simulink model "afe_inv_psm_param"  (R2026b)
settings: Solver=ode23t  StopTime=param.sim.simlength  FixedStep=tc  MaxStep=param.glb_time.tc  RelTol=1e-4
values from neighbouring files (symbols this model uses):
  param = add_template_extras(param, options)    [init_model.m]
undefined symbols (not defined in the file or in its folder): magnitude, omega_m_bez
libraries: fl_lib x330, nesl_utility x174, igbt_simple_2th_lib x12, moving_average_filter x10, moving_average_filter_cc x8, sl_discontinuities x3, single_phase_transformer_lib x3, linear_double_integrator_observer_ccaller x2, discrete_time_low_pass_filter x2, threephase_inductor_lib x2, three_phase_pwm_modulator x2, three_phase_inverter_ideal_switch_based_model x2
(part 3 of 13)

== system afe_inv_psm_param/afe_abc_inv_psm_mod1/afe/three_phase_inverter_igbt_based_with_thermal_model ==
  gate_commands : Inport
  Bus Selector : BusSelector  OutputSignals=module_1.igbt_ploss_Q2,module_1.igbt_voltage_Q2,module_1.igbt_current_Q2,module_1.igbt_JH_temp_Q2,module_1.igbt_HA_temp_Q2
  Bus Selector1 : BusSelector  OutputSignals=module_1.igbt_ploss_Q1,module_1.igbt_voltage_Q1,module_1.igbt_current_Q1,module_1.igbt_JH_temp_Q1,module_1.igbt_HA_temp_Q1
  Bus Selector2 : BusSelector  OutputSignals=module_2.igbt_ploss_Q3,module_2.igbt_voltage_Q3,module_2.igbt_current_Q3,module_2.igbt_JH_temp_Q3,module_2.igbt_HA_temp_Q3
  Bus Selector3 : BusSelector  OutputSignals=module_1.diode_ploss_Q1,module_1.diode_JH_temp_Q1,module_1.diode_HA_temp_Q1,module_1.diode_current_Q1
  three_phase_inverter_with_igbt_simple_2th : Subsystem  mask{vce_sat_m=param.afe.igbt.Vce_sat, v_gamma_m=param.afe.igbt.Vdon_diode, Vth_gate_m=param.afe.igbt.Vth, Vth_gate_hyst_m=0.85, Eon_m=param.afe.igbt.Eon*1000, Eoff_m=param.afe.igbt.Eoff*1000, Err_m=param.afe.igbt.Erec*1000, Ic_ref_m=param.afe.igbt.Ion_sw_losses, Vdc_ref_m=param.afe.igbt.Voff_sw_losses, Vblock_Errf_m=50, rce_on_m=param.afe.igbt.Rce_on*1000, rd_on_m=param.afe.igbt.Rdon_diode*1000, Gce_off_m=1e-6, time_constant_edge_m=param.glb_time.tc, time_constant_ploss_m=1e3, Csnubber_m=param.afe.igbt.Csnubber, Rsnubber_m=param.afe.igbt.Rsnubber, rth_switch_JH_m=param.afe.igbt.Rth_switch_JH, rth_switch_HA_m=param.thermal.heatsink.Rth_switch_HA, rth_diode_JH_m=param.afe.igbt.Rth_diode_JH, rth_diode_HA_m=param.thermal.heatsink.Rth_diode_HA, JunctionTermalMass_m=param.afe.igbt.JunctionTermalMass, Tambient_m=param.thermal.Tambient, mass_heatsink_m=param.thermal.heatsink.no_weight, specific_heat_m=param.thermal.heatsink.cp}
      mask prompts: vce_sat_m "Collector-emitter on-stage voltage [V]"; v_gamma_m "Diode forward voltage [V]"; Vth_gate_m "Gate-emitter threshold voltage [V]"; Vth_gate_hyst_m "Half hysteresis band for the switching events [V]"; Eon_m "Turn-on energy at Ic_ref, Vdc_ref [mJ]"; Eoff_m "Turn-off energy at Ic_ref, Vdc_ref [mJ]"; Err_m "Reverse recovery energy at Ic_ref, Vdc_ref [mJ]"; Ic_ref_m "Reference current of the energies [A]"; Vdc_ref_m "Reference voltage of the energies [V]"; Vblock_Errf_m "V block Err"; rce_on_m "IGBT on-state series resistance [mOhm]"; rd_on_m "Diode series resistance [mOhm]"; Gce_off_m "Off-state conductance [1/Ohm]"; time_constant_edge_m "Sample&hold time constant (<< on-time) [us]"; time_constant_ploss_m "Loss averaging time constant (2-5 x Tsw) [us]"; Csnubber_m "Csnubber [F]"; Rsnubber_m "Rsnubber [Ohm]"; rth_switch_JH_m "Thermal impedance Junction-heatsink switch [K/W]"; rth_switch_HA_m "Thermal impedance heatsink-ambient switch[K/W]"; rth_diode_JH_m "Thermal impedance Junction-heatsink diode [K/W]"; rth_diode_HA_m "Thermal impedance heatsink-ambient diode [K/W]"; JunctionTermalMass_m "Junction Thermal Mass [J/K]"; Tambient_m "Ambient temperature [degC]"; mass_heatsink_m "Mass heatsink [kg]"; specific_heat_m "Specific heat capacity of the heatsink [J/K/Kg]"
  udc(+) : PMIOPort  Side=Left
  u : PMIOPort  Port=2  Side=Right
  v : PMIOPort  Port=3  Side=Right
  udc(-) : PMIOPort  Port=4  Side=Left
  w : PMIOPort  Port=5  Side=Right
  tag scope: diode_HA_temp_afeQ1=global, diode_JH_temp_afeQ1=global, diode_current_afeQ1=global, diode_ploss_afeQ1=global, igbt_HA_temp_afeQ1=global, igbt_HA_temp_afeQ2=global, igbt_HA_temp_afeQ3=global, igbt_JH_temp_afeQ1=global, igbt_JH_temp_afeQ2=global, igbt_JH_temp_afeQ3=global, igbt_current_afeQ1=global, igbt_current_afeQ2=global, igbt_current_afeQ3=global, igbt_ploss_afeQ1=global, igbt_ploss_afeQ2=global, igbt_ploss_afeQ3=global, igbt_voltage_afeQ1=global, igbt_voltage_afeQ2=global, igbt_voltage_afeQ3=global
  wires:
  gate_commands/1 -> three_phase_inverter_with_igbt_simple_2th/1(gate_commands)
  Bus Selector3/3 -> [diode_HA_temp_afeQ1]  "<diode_HA_temp_Q1>"
  Bus Selector/1 -> [igbt_ploss_afeQ2]  "<igbt_ploss_Q2>"
  Bus Selector3/2 -> [diode_JH_temp_afeQ1]  "<diode_JH_temp_Q1>"
  Bus Selector1/2 -> [igbt_voltage_afeQ1]  "<igbt_voltage_Q1>"
  Bus Selector/2 -> [igbt_voltage_afeQ2]  "<igbt_voltage_Q2>"
  Bus Selector/5 -> [igbt_HA_temp_afeQ2]  "<igbt_HA_temp_Q2>"
  Bus Selector2/5 -> [igbt_HA_temp_afeQ3]  "<igbt_HA_temp_Q3>"
  Bus Selector2/2 -> [igbt_voltage_afeQ3]  "<igbt_voltage_Q3>"
  Bus Selector/4 -> [igbt_JH_temp_afeQ2]  "<igbt_JH_temp_Q2>"
  Bus Selector1/4 -> [igbt_JH_temp_afeQ1]  "<igbt_JH_temp_Q1>"
  Bus Selector3/1 -> [diode_ploss_afeQ1]  "<diode_ploss_Q1>"
  Bus Selector2/4 -> [igbt_JH_temp_afeQ3]  "<igbt_JH_temp_Q3>"
  Bus Selector2/3 -> [igbt_current_afeQ3]  "<igbt_current_Q3>"
  three_phase_inverter_with_igbt_simple_2th/1(m) -> Bus Selector3/1, Bus Selector2/1, Bus Selector/1, Bus Selector1/1
  Bus Selector1/3 -> [igbt_current_afeQ1]  "<igbt_current_Q1>"
  Bus Selector/3 -> [igbt_current_afeQ2]  "<igbt_current_Q2>"
  Bus Selector1/5 -> [igbt_HA_temp_afeQ1]  "<igbt_HA_temp_Q1>"
  Bus Selector2/1 -> [igbt_ploss_afeQ3]  "<igbt_ploss_Q3>"
  Bus Selector1/1 -> [igbt_ploss_afeQ1]  "<igbt_ploss_Q1>"
  Bus Selector3/4 -> [diode_current_afeQ1]  "<diode_current_Q1>"
  connections:
  u/RConn1 -- three_phase_inverter_with_igbt_simple_2th/RConn1
  v/RConn1 -- three_phase_inverter_with_igbt_simple_2th/RConn2
  udc(-)/RConn1 -- three_phase_inverter_with_igbt_simple_2th/LConn2
  udc(+)/RConn1 -- three_phase_inverter_with_igbt_simple_2th/LConn1
  w/RConn1 -- three_phase_inverter_with_igbt_simple_2th/RConn3

== system afe_inv_psm_param/afe_abc_inv_psm_mod1/afe/three_phase_inverter_mosfet_based_with_thermal_model ==
  gate_commands : Inport
  Bus Selector : BusSelector  OutputSignals=mosfet_ploss_Q2,mosfet_voltage_Q2,mosfet_current_Q2,mosfet_JH_temp_Q2,mosfet_HA_temp_Q2
  Bus Selector1 : BusSelector  OutputSignals=mosfet_ploss_Q1,mosfet_voltage_Q1,mosfet_current_Q1,mosfet_JH_temp_Q1,mosfet_HA_temp_Q1
  Bus Selector2 : BusSelector  OutputSignals=mosfet_ploss_Q3,mosfet_voltage_Q3,mosfet_current_Q3,mosfet_JH_temp_Q3,mosfet_HA_temp_Q3
  three phase inverter mosfet based with thermal model : three_phase_inverter_mosfet_based_with_thermal_model/three phase inverter mosfet based with thermal model  mass_heatsink_m=0.2  specific_heat_m=880  rth_mosfet_HA_m=0.02  rth_mosfet_JH_m=0.075  Rds_on_m=0.00185  Vth_m=7.5  Eon_m=0.077  Eoff_m=0.108  Voff_sw_loss_m=1300  Ion_sw_loss_m=1000  Vdon_diode_m=4  Rdon_diode_m=0.00185  JunctionTermalMass_m=2  Tambient_m=40  DThs_init_m=0
  u : PMIOPort  Side=Right
  udc(+) : PMIOPort  Port=2  Side=Left
  v : PMIOPort  Port=3  Side=Right
  udc(-) : PMIOPort  Port=4  Side=Left
  w : PMIOPort  Port=5  Side=Right
  tag scope: mosfet_HA_temp_afeQ1=global, mosfet_HA_temp_afeQ2=global, mosfet_HA_temp_afeQ3=global, mosfet_JH_temp_afeQ1=global, mosfet_JH_temp_afeQ2=global, mosfet_JH_temp_afeQ3=global, mosfet_current_afeQ1=global, mosfet_current_afeQ2=global, mosfet_current_afeQ3=global, mosfet_ploss_afeQ1=global, mosfet_ploss_afeQ2=global, mosfet_ploss_afeQ3=global, mosfet_voltage_afeQ1=global, mosfet_voltage_afeQ2=global, mosfet_voltage_afeQ3=global
  wires:
  gate_commands/1 -> three phase inverter mosfet based with thermal model/1
  three phase inverter mosfet based with thermal model/1 -> Bus Selector/1, Bus Selector2/1, Bus Selector1/1
  Bus Selector2/1 -> [mosfet_ploss_afeQ3]  "<mosfet_ploss_Q3>"
  Bus Selector2/2 -> [mosfet_voltage_afeQ3]  "<mosfet_voltage_Q3>"
  Bus Selector2/3 -> [mosfet_current_afeQ3]  "<mosfet_current_Q3>"
  Bus Selector2/5 -> [mosfet_HA_temp_afeQ3]  "<mosfet_HA_temp_Q3>"
  Bus Selector2/4 -> [mosfet_JH_temp_afeQ3]  "<mosfet_JH_temp_Q3>"
  Bus Selector/1 -> [mosfet_ploss_afeQ2]  "<mosfet_ploss_Q2>"
  Bus Selector/2 -> [mosfet_voltage_afeQ2]  "<mosfet_voltage_Q2>"
  Bus Selector/3 -> [mosfet_current_afeQ2]  "<mosfet_current_Q2>"
  Bus Selector/4 -> [mosfet_JH_temp_afeQ2]  "<mosfet_JH_temp_Q2>"
  Bus Selector/5 -> [mosfet_HA_temp_afeQ2]  "<mosfet_HA_temp_Q2>"
  Bus Selector1/1 -> [mosfet_ploss_afeQ1]  "<mosfet_ploss_Q1>"
  Bus Selector1/2 -> [mosfet_voltage_afeQ1]  "<mosfet_voltage_Q1>"
  Bus Selector1/3 -> [mosfet_current_afeQ1]  "<mosfet_current_Q1>"
  Bus Selector1/4 -> [mosfet_JH_temp_afeQ1]  "<mosfet_JH_temp_Q1>"
  Bus Selector1/5 -> [mosfet_HA_temp_afeQ1]  "<mosfet_HA_temp_Q1>"
  connections:
  three phase inverter mosfet based with thermal model/RConn3 -- w/RConn1
  three phase inverter mosfet based with thermal model/RConn2 -- v/RConn1
  three phase inverter mosfet based with thermal model/LConn1 -- udc(+)/RConn1
  three phase inverter mosfet based with thermal model/LConn2 -- udc(-)/RConn1
  three phase inverter mosfet based with thermal model/RConn1 -- u/RConn1

== system afe_inv_psm_param/afe_abc_inv_psm_mod1/battery/single_phase_ui_measure ==
  Bus Creator : BusCreator  Inputs=2
  Current Sensor : fl_lib/Electrical/Electrical Sensors/Current Sensor
  Selector : Selector  InputPortWidth=2  IndexOptions=Index vector (dialog)  Indices=2  OutputSizes=1  RuntimeRangeChecks=off
  Selector1 : Selector  InputPortWidth=2  IndexOptions=Index vector (dialog)  Indices=1  OutputSizes=1  RuntimeRangeChecks=off
  Voltage Sensor : fl_lib/Electrical/Electrical Sensors/Voltage Sensor
  dab input modA : Scope  NumInputPorts=2
      settings: ActiveDisplayYMinimum=-413.54291450338707  ActiveDisplayYMaximum=396.93489435257015  DataLoggingVariableName=ScopeData2
  iph : nesl_utility/PS-Simulink Converter  PhysicalDomain=network_engine_domain  SubClassName=ps_output  LeftPortType=input  RightPortType=output  PseudoPeriodic=off  Frequencies=[]  VectorFormat=1-D array  Unit=A  AffineConversion=off
  uph : nesl_utility/PS-Simulink Converter  PhysicalDomain=network_engine_domain  SubClassName=ps_output  LeftPortType=input  RightPortType=output  PseudoPeriodic=off  Frequencies=[]  VectorFormat=1-D array  Unit=V  AffineConversion=off
  Udc(+) : PMIOPort  Side=Left
  udc(+) : PMIOPort  Port=2  Side=Right
  Udc(-) : PMIOPort  Port=3  Side=Left
  udc(-) : PMIOPort  Port=4  Side=Right
  tag scope: current_battery=global, voltage_battery=global
  wires:
  Bus Creator/1 -> Selector/1, Selector1/1  "ui_data"
  iph/1 -> Bus Creator/1  "iph"
  uph/1 -> Bus Creator/2  "uph"
  Selector1/1 -> [current_battery], dab input modA/1  "current_battery"
  Selector/1 -> dab input modA/2, [voltage_battery]  "voltage_battery"
  connections:
  iph/LConn1 -- Current Sensor/RConn1
  Voltage Sensor/LConn1 -- Current Sensor/LConn1 -- Udc(+)/RConn1
  Current Sensor/RConn2 -- udc(+)/RConn1
  Voltage Sensor/RConn1 -- uph/LConn1
  Voltage Sensor/RConn2 -- Udc(-)/RConn1 -- udc(-)/RConn1

== system afe_inv_psm_param/afe_abc_inv_psm_mod1/brake/Rbrake ==
  PS-Simulink Converter2 : nesl_utility/PS-Simulink Converter  PhysicalDomain=network_engine_domain  SubClassName=ps_output  LeftPortType=input  RightPortType=output  PseudoPeriodic=off  Frequencies=[]  VectorFormat=1-D array  Unit=degC  AffineConversion=off
  PS-Simulink Converter3 : nesl_utility/PS-Simulink Converter  PhysicalDomain=network_engine_domain  SubClassName=ps_output  LeftPortType=input  RightPortType=output  PseudoPeriodic=off  Frequencies=[]  VectorFormat=1-D array  Unit=W  AffineConversion=off
  Rbrake_thermal : Scope  NumInputPorts=2
      settings: ActiveDisplayYMinimum=-0.005623823950706707  ActiveDisplayYMaximum=0.05061441555636037  DataLoggingVariableName=ScopeData33
  Resistor1 : ee_lib/Passive/Resistor  R=param.afe.hw.Rbrake Ohm  enable_R_tol=ee.enum.toleranceApplication.none  R_tol=5  tol_distribution=ee.enum.toleranceDistribution.uniform  nSigma=4  enable_operating_limits=ee.enum.enable.no  operating_limit_action=ee.enum.passive.reportOpLim.warn  power_rating=1 W  max_working_voltage=100 V  noise_mode=ee.enum.sources.noise.Disabled  Tdevice=25 degC  sample_time=1e-3 s  repeatability=ee.enum.ic.repeatability.notRepeatable  user_seed=0  auto_seed=3499211588  power_derating_T1=70 degC  power_derating_T2=155 degC  operating_temperature_range_vec=[-50, 150] degC  alpha=3.93e-3 1/K  Tmeas=25 degC  thermal_mass=100 J/K  temperature_specify=off  temperature_priority=High  temperature=298.15 K  temperature_nominal_specify=off  temperature_nominal_value=1  temperature_nominal_unit=K
  Tambient : fl_lib/Thermal/Thermal Sources/Temperature Source  temperature=param.thermal.Tambient degC
  Temperature Sensor1 : fl_lib/Thermal/Thermal Sensors/Temperature Sensor  temperature_measure=foundation.enum.MeasurementReference.difference
  To Workspace1 : ToWorkspace  VariableName=RbrakePowerFlow_mod1_sim  SampleTime=param.glb_time.tc
      settings: MaxDataPoints=param.glb_time.Nc
  To Workspace10 : ToWorkspace  VariableName=RbrakeTemperature_mod1_sim  SampleTime=param.glb_time.tc
      settings: MaxDataPoints=param.glb_time.Nc
  heatsink_C : fl_lib/Thermal/Thermal Elements/Thermal Mass  mass_type=foundation.enum.constant_variable.constant  mass=40 kg  sp_heat=505 J/(K*kg)  mass_min=1e-6 kg  num_ports=foundation.enum.numPorts2.one  m_specify=off  m_priority=High  m=1 kg  m_nominal_specify=off  m_nominal_value=1  m_nominal_unit=kg  T_specify=on  T_priority=High  T=param.thermal.DThs_init+param.thermal.Tambient degC  T_nominal_specify=off  T_nominal_value=1  T_nominal_unit=K  Q_specify=off  Q_priority=High  Q=0 W  Q_nominal_specify=off  Q_nominal_value=1  Q_nominal_unit=W
  power_losses_switch : fl_lib/Thermal/Thermal Sensors/Heat Flow Rate Sensor
  switch_heatsink : fl_lib/Thermal/Thermal Elements/Thermal Resistance  resistance=300/48e3 K/W  T_specify=off  T_priority=High  T=0 deltadegC  T_nominal_specify=off  T_nominal_value=1  T_nominal_unit=K  Q_specify=off  Q_priority=None  Q=0 W  Q_nominal_specify=off  Q_nominal_value=1  Q_nominal_unit=W
  A : PMIOPort  Side=Left
  B : PMIOPort  Port=2  Side=Right
  wires:
  PS-Simulink Converter2/1 -> To Workspace10/1, Rbrake_thermal/1  "RbrakeTemperature"
  PS-Simulink Converter3/1 -> To Workspace1/1, Rbrake_thermal/2  "RbrakePowerFlow"
  connections:
  Resistor1/LConn1 -- A/RConn1
  Resistor1/RConn1 -- B/RConn1
  Tambient/LConn1 -- Temperature Sensor1/RConn1 -- switch_heatsink/RConn1
  Temperature Sensor1/LConn1 -- power_losses_switch/RConn2 -- heatsink_C/LConn1 -- switch_heatsink/LConn1
  Temperature Sensor1/RConn2 -- PS-Simulink Converter2/LConn1
  power_losses_switch/LConn1 -- Resistor1/LConn2
  power_losses_switch/RConn1 -- PS-Simulink Converter3/LConn1

== system afe_inv_psm_param/afe_abc_inv_psm_mod1/brake/switch_1 ==
  Capacitor : fl_lib/Electrical/Electrical Elements/Capacitor  c=param.afe.ideal_switch.Csnubber F  r=param.afe.ideal_switch.Rsnubber Ohm  g=0 1/Ohm  i_specify=off  i_priority=None  i=0 A  i_nominal_specify=off  i_nominal_value=1  i_nominal_unit=A  v_specify=off  v_priority=None  v=0 V  v_nominal_specify=off  v_nominal_value=1  v_nominal_unit=V  vc_specify=off  vc_priority=High  vc=0 V  vc_nominal_specify=off  vc_nominal_value=1  vc_nominal_unit=V
  Diode : fl_lib/Electrical/Electrical Elements/Diode  Vf=param.afe.ideal_switch.Vgamma V  Ron=param.afe.ideal_switch.Rdon_diode Ohm  Goff=1e-8 1/Ohm  i_specify=off  i_priority=None  i=0 A  i_nominal_specify=off  i_nominal_value=1  i_nominal_unit=A  v_specify=off  v_priority=None  v=0 V  v_nominal_specify=off  v_nominal_value=1  v_nominal_unit=V
  C : PMIOPort  Side=Left
  E : PMIOPort  Port=2  Side=Right
  connections:
  Diode/LConn1 -- Capacitor/RConn1 -- E/RConn1
  Diode/RConn1 -- C/RConn1 -- Capacitor/LConn1

== system afe_inv_psm_param/afe_abc_inv_psm_mod1/brake/switch_2 ==
  Capacitor : fl_lib/Electrical/Electrical Elements/Capacitor  c=param.afe.ideal_switch.Csnubber F  r=param.afe.ideal_switch.Rsnubber Ohm  g=0 1/Ohm  i_specify=off  i_priority=None  i=0 A  i_nominal_specify=off  i_nominal_value=1  i_nominal_unit=A  v_specify=off  v_priority=None  v=0 V  v_nominal_specify=off  v_nominal_value=1  v_nominal_unit=V  vc_specify=off  vc_priority=High  vc=0 V  vc_nominal_specify=off  vc_nominal_value=1  vc_nominal_unit=V
  Diode : fl_lib/Electrical/Electrical Elements/Diode  Vf=param.afe.ideal_switch.Vgamma V  Ron=param.afe.ideal_switch.Rdon_diode Ohm  Goff=1e-8 1/Ohm  i_specify=off  i_priority=None  i=0 A  i_nominal_specify=off  i_nominal_value=1  i_nominal_unit=A  v_specify=off  v_priority=None  v=0 V  v_nominal_specify=off  v_nominal_value=1  v_nominal_unit=V
  Switch : fl_lib/Electrical/Electrical Elements/Switch  R_closed=param.afe.ideal_switch.Rds_on Ohm  G_open=1e-8 1/Ohm  Threshold=7.5  i_specify=off  i_priority=None  i=0 A  i_nominal_specify=off  i_nominal_value=1  i_nominal_unit=A  v_specify=off  v_priority=None  v=0 V  v_nominal_specify=off  v_nominal_value=1  v_nominal_unit=V
  G : PMIOPort  Side=Left
  C : PMIOPort  Port=2  Side=Left
  E : PMIOPort  Port=3  Side=Right
  connections:
  Switch/RConn2 -- C/RConn1 -- Capacitor/LConn1 -- Diode/RConn1
  Switch/RConn1 -- G/RConn1
  Switch/LConn1 -- E/RConn1 -- Capacitor/RConn1 -- Diode/LConn1

== system afe_inv_psm_param/afe_abc_inv_psm_mod1/inverter/inverter ==
  gate_cmds_uvw : Inport
  sv_pwm : Subsystem
  three_phase_inverter_ideal_switch_based_model : Subsystem  Commented=on
  three_phase_inverter_igbt_based_with_thermal_model : Subsystem
  three_phase_inverter_mosfet_based_with_thermal_model : Subsystem  Commented=on
  u : PMIOPort  Side=Left
  v : PMIOPort  Port=2  Side=Left
  w : PMIOPort  Port=3  Side=Left
  udc(+) : PMIOPort  Port=4  Side=Right
  udc(-) : PMIOPort  Port=5  Side=Right
  wires:
  sv_pwm/1(gate_cmds) -> three_phase_inverter_mosfet_based_with_thermal_model/1(gate_commands), three_phase_inverter_igbt_based_with_thermal_model/1(gate_commands), three_phase_inverter_ideal_switch_based_model/1(gate_commands)
  gate_cmds_uvw/1 -> sv_pwm/1(gate_cmds_uvw)
  connections:
  udc(+)/RConn1 -- three_phase_inverter_ideal_switch_based_model/LConn1 -- three_phase_inverter_igbt_based_with_thermal_model/LConn1 -- three_phase_inverter_mosfet_based_with_thermal_model/LConn1
  udc(-)/RConn1 -- three_phase_inverter_ideal_switch_based_model/LConn2 -- three_phase_inverter_igbt_based_with_thermal_model/LConn2 -- three_phase_inverter_mosfet_based_with_thermal_model/LConn2
  u/RConn1 -- three_phase_inverter_igbt_based_with_thermal_model/RConn1 -- three_phase_inverter_ideal_switch_based_model/RConn1 -- three_phase_inverter_mosfet_based_with_thermal_model/RConn1
  v/RConn1 -- three_phase_inverter_igbt_based_with_thermal_model/RConn2 -- three_phase_inverter_ideal_switch_based_model/RConn2 -- three_phase_inverter_mosfet_based_with_thermal_model/RConn2
  w/RConn1 -- three_phase_inverter_igbt_based_with_thermal_model/RConn3 -- three_phase_inverter_ideal_switch_based_model/RConn3 -- three_phase_inverter_mosfet_based_with_thermal_model/RConn3

== system afe_inv_psm_param/grid/grid_emulator/3ph_Dyg ==
  Electrical Reference1 : fl_lib/Electrical/Electrical Elements/Electrical Reference
  ph1 : single_phase_transformer_lib/single phase transformer  Lm=param.grid.emu.trafo.Lm1 H  n1=param.grid.emu.trafo.n1  n2=param.grid.emu.trafo.n2  Rd1=param.grid.emu.trafo.Rd1 Ohm  Rd2=param.grid.emu.trafo.Rd2 Ohm  Ld1=param.grid.emu.trafo.Ld1 H  Ld2=param.grid.emu.trafo.Ld2 H  Rfe=param.grid.emu.trafo.Rfe1 Ohm  phi_specify=off  phi_priority=None  phi=0 V*s  phi_nominal_specify=off  phi_nominal_value=1  phi_nominal_unit=V*s  i1_specify=off  i1_priority=None  i1=0 A  i1_nominal_specify=off  i1_nominal_value=1  i1_nominal_unit=A  i2_specify=off  i2_priority=None  i2=0 A  i2_nominal_specify=off  i2_nominal_value=1  i2_nominal_unit=A  ife_specify=off  ife_priority=None  ife=0 A  ife_nominal_specify=off  ife_nominal_value=1  ife_nominal_unit=A  u1_specify=off  u1_priority=None  u1=0 V  u1_nominal_specify=off  u1_nominal_value=1  u1_nominal_unit=V  u2_specify=off  u2_priority=None  u2=0 V  u2_nominal_specify=off  u2_nominal_value=1  u2_nominal_unit=V
  ph2 : single_phase_transformer_lib/single phase transformer  Lm=param.grid.emu.trafo.Lm1 H  n1=param.grid.emu.trafo.n1  n2=param.grid.emu.trafo.n2  Rd1=param.grid.emu.trafo.Rd1 Ohm  Rd2=param.grid.emu.trafo.Rd2 Ohm  Ld1=param.grid.emu.trafo.Ld1 H  Ld2=param.grid.emu.trafo.Ld2 H  Rfe=param.grid.emu.trafo.Rfe1 Ohm  phi_specify=off  phi_priority=None  phi=0 V*s  phi_nominal_specify=off  phi_nominal_value=1  phi_nominal_unit=V*s  i1_specify=off  i1_priority=None  i1=0 A  i1_nominal_specify=off  i1_nominal_value=1  i1_nominal_unit=A  i2_specify=off  i2_priority=None  i2=0 A  i2_nominal_specify=off  i2_nominal_value=1  i2_nominal_unit=A  ife_specify=off  ife_priority=None  ife=0 A  ife_nominal_specify=off  ife_nominal_value=1  ife_nominal_unit=A  u1_specify=off  u1_priority=None  u1=0 V  u1_nominal_specify=off  u1_nominal_value=1  u1_nominal_unit=V  u2_specify=off  u2_priority=None  u2=0 V  u2_nominal_specify=off  u2_nominal_value=1  u2_nominal_unit=V
  ph3 : single_phase_transformer_lib/single phase transformer  Lm=param.grid.emu.trafo.Lm1 H  n1=param.grid.emu.trafo.n1  n2=param.grid.emu.trafo.n2  Rd1=param.grid.emu.trafo.Rd1 Ohm  Rd2=param.grid.emu.trafo.Rd2 Ohm  Ld1=param.grid.emu.trafo.Ld1 H  Ld2=param.grid.emu.trafo.Ld2 H  Rfe=param.grid.emu.trafo.Rfe1 Ohm  phi_specify=off  phi_priority=None  phi=0 V*s  phi_nominal_specify=off  phi_nominal_value=1  phi_nominal_unit=V*s  i1_specify=off  i1_priority=None  i1=0 A  i1_nominal_specify=off  i1_nominal_value=1  i1_nominal_unit=A  i2_specify=off  i2_priority=None  i2=0 A  i2_nominal_specify=off  i2_nominal_value=1  i2_nominal_unit=A  ife_specify=off  ife_priority=None  ife=0 A  ife_nominal_specify=off  ife_nominal_value=1  ife_nominal_unit=A  u1_specify=off  u1_priority=None  u1=0 V  u1_nominal_specify=off  u1_nominal_value=1  u1_nominal_unit=V  u2_specify=off  u2_priority=None  u2=0 V  u2_nominal_specify=off  u2_nominal_value=1  u2_nominal_unit=V
  ua : PMIOPort  Side=Right
  ub : PMIOPort  Port=2  Side=Right
  uc : PMIOPort  Port=3  Side=Right
  Ua : PMIOPort  Port=4  Side=Left
  Ub : PMIOPort  Port=5  Side=Left
  Uc : PMIOPort  Port=6  Side=Left
  connections:
  Electrical Reference1/LConn1 -- ph3/RConn2 -- ph2/RConn2 -- ph1/RConn2
  ph3/RConn1 -- uc/RConn1
  ph1/LConn1 -- ph3/LConn2 -- Ua/RConn1
  ph1/RConn1 -- ua/RConn1
  ph2/RConn1 -- ub/RConn1
  ph1/LConn2 -- ph2/LConn1 -- Ub/RConn1
  Uc/RConn1 -- ph3/LConn1 -- ph2/LConn2

== system afe_inv_psm_param/grid/grid_emulator/threephase_vi_measures ==
  Bus Creator : BusCreator  Inputs=6
  Current Sensor : fl_lib/Electrical/Electrical Sensors/Current Sensor
  Current Sensor1 : fl_lib/Electrical/Electrical Sensors/Current Sensor
  Current Sensor2 : fl_lib/Electrical/Electrical Sensors/Current Sensor
  Electrical Reference1 : fl_lib/Electrical/Electrical Elements/Electrical Reference
  Voltage Sensor : fl_lib/Electrical/Electrical Sensors/Voltage Sensor
  Voltage Sensor1 : fl_lib/Electrical/Electrical Sensors/Voltage Sensor
  Voltage Sensor2 : fl_lib/Electrical/Electrical Sensors/Voltage Sensor
  i : Selector  InputPortWidth=6  IndexOptions=Index vector (dialog)  Indices=[4 5 6]  OutputSizes=1  RuntimeRangeChecks=off
  ia_grid : nesl_utility/PS-Simulink Converter  PhysicalDomain=network_engine_domain  SubClassName=ps_output  LeftPortType=input  RightPortType=output  PseudoPeriodic=off  Frequencies=[]  VectorFormat=1-D array  Unit=A  AffineConversion=off
  ib_grid : nesl_utility/PS-Simulink Converter  PhysicalDomain=network_engine_domain  SubClassName=ps_output  LeftPortType=input  RightPortType=output  PseudoPeriodic=off  Frequencies=[]  VectorFormat=1-D array  Unit=A  AffineConversion=off
  ic_grid : nesl_utility/PS-Simulink Converter  PhysicalDomain=network_engine_domain  SubClassName=ps_output  LeftPortType=input  RightPortType=output  PseudoPeriodic=off  Frequencies=[]  VectorFormat=1-D array  Unit=A  AffineConversion=off
  u : Selector  InputPortWidth=6  IndexOptions=Index vector (dialog)  Indices=[1 2 3]  OutputSizes=1  RuntimeRangeChecks=off
  ua_grid : nesl_utility/PS-Simulink Converter  PhysicalDomain=network_engine_domain  SubClassName=ps_output  LeftPortType=input  RightPortType=output  PseudoPeriodic=off  Frequencies=[]  VectorFormat=1-D array  Unit=V  AffineConversion=off
  ub_grid : nesl_utility/PS-Simulink Converter  PhysicalDomain=network_engine_domain  SubClassName=ps_output  LeftPortType=input  RightPortType=output  PseudoPeriodic=off  Frequencies=[]  VectorFormat=1-D array  Unit=V  AffineConversion=off
  uc_grid : nesl_utility/PS-Simulink Converter  PhysicalDomain=network_engine_domain  SubClassName=ps_output  LeftPortType=input  RightPortType=output  PseudoPeriodic=off  Frequencies=[]  VectorFormat=1-D array  Unit=V  AffineConversion=off
  Ua : PMIOPort  Side=Left
  ua : PMIOPort  Port=2  Side=Right
  Ub : PMIOPort  Port=3  Side=Left
  ub : PMIOPort  Port=4  Side=Right
  Uc : PMIOPort  Port=5  Side=Left
  uc : PMIOPort  Port=6  Side=Right
  tag scope: i_abc_line=global, u_abc_line=global
  wires:
  Bus Creator/1 -> i/1, u/1  "vi_data"
  ib_grid/1 -> Bus Creator/5  "ib"
  ia_grid/1 -> Bus Creator/4  "ia"
  ic_grid/1 -> Bus Creator/6  "ic"
  ua_grid/1 -> Bus Creator/1  "ua"
  ub_grid/1 -> Bus Creator/2  "ub"
  uc_grid/1 -> Bus Creator/3  "uc"
  i/1 -> [i_abc_line]
  u/1 -> [u_abc_line]
  connections:
  Current Sensor1/LConn1 -- Ub/RConn1 -- Voltage Sensor1/LConn1
  Electrical Reference1/LConn1 -- Voltage Sensor/RConn2 -- Voltage Sensor2/RConn2 -- Voltage Sensor1/RConn2
  Voltage Sensor/RConn1 -- ua_grid/LConn1
  Current Sensor/RConn2 -- ua/RConn1
  Voltage Sensor1/RConn1 -- ub_grid/LConn1
  Voltage Sensor2/LConn1 -- Current Sensor2/LConn1 -- Uc/RConn1
  Current Sensor/LConn1 -- Ua/RConn1 -- Voltage Sensor/LConn1
  Current Sensor1/RConn2 -- ub/RConn1
  Voltage Sensor2/RConn1 -- uc_grid/LConn1
  ib_grid/LConn1 -- Current Sensor1/RConn1
  ia_grid/LConn1 -- Current Sensor/RConn1
  ic_grid/LConn1 -- Current Sensor2/RConn1
  Current Sensor2/RConn2 -- uc/RConn1

== system afe_inv_psm_param/afe_abc_inv_psm_mod1/AFE_control/afe_control/FRT-VDE4110 ==
  Constant : Constant  Value=0
  FRT-Detection : Subsystem
  FRT-PosNegReactiveCurrentReferences : Subsystem
  Terminator : Terminator
  Terminator1 : Terminator
  frt_detection_output : Scope  NumInputPorts=3
      settings: ActiveDisplayYMinimum=-0.12499999999999997  ActiveDisplayYMaximum=1.125
  tag scope: frt_active=scoped, pwr_lim_enable=scoped
  wires:
  [v_grid_pos_xi_avg] -> FRT-PosNegReactiveCurrentReferences/1(In1)
  [v_grid_neg_xi_avg] -> FRT-PosNegReactiveCurrentReferences/3(In3)
  [v_grid_neg_eta_avg] -> FRT-PosNegReactiveCurrentReferences/4(In4)
  [v_grid_pos_eta_avg] -> FRT-PosNegReactiveCurrentReferences/2(In2)
  FRT-Detection/4(frt_active) -> frt_detection_output/2, [frt_active]  "frt_active"
  FRT-Detection/5(pwr_lim_enable) -> frt_detection_output/3, [pwr_lim_enable]  "pwr_lim_enable"
  FRT-Detection/2(frt_state) -> frt_detection_output/1  "frt_state"
  Constant/1 -> FRT-Detection/1(red_dyn_enabled)
  FRT-Detection/1(frt_exceeded) -> Terminator/1
  FRT-Detection/3(red_dyn_active) -> Terminator1/1

== system afe_inv_psm_param/afe_abc_inv_psm_mod1/AFE_control/afe_control/current_ctrl ==
  i_xi_ref : Inport
  Demux : Demux  Outputs=3
  current_transformation : Subsystem
  inner_current_ctrl : Subsystem
  xieta2abc_ref : Subsystem
  u_alpha_beta_gamma_out : Outport
  wires:
  Demux/1 -> current_transformation/1(is_a_pu)  "is_a"
  Demux/2 -> current_transformation/2(is_b_pu)  "is_b"
  Demux/3 -> current_transformation/3(is_c_pu)  "is_c"
  [isd_abc_pu] -> Demux/1
  [phase_grid_pll] -> xieta2abc_ref/5(phase)
  xieta2abc_ref/1(i_abc_ref) -> inner_current_ctrl/1(In1)
  [isd_abc_pu] -> inner_current_ctrl/2(is_abc)
  inner_current_ctrl/1(uabg) -> u_alpha_beta_gamma_out/1
  i_xi_ref/1 -> xieta2abc_ref/1(pos_xi_ref)  "i_xi_ref"
  [i_stack_neg_eta_ref] -> xieta2abc_ref/4(neg_eta)
  [i_stack_neg_xi_ref] -> xieta2abc_ref/3(neg_xi)
  [i_stack_pos_eta_ref] -> xieta2abc_ref/2(pos_eta)

== system afe_inv_psm_param/afe_abc_inv_psm_mod1/AFE_control/afe_control/data_to_worspace_module_1 ==
  Bus Creator : BusCreator  Inputs=5
  dq_pll : Subsystem
  inner_current_tracking : Subsystem
  pwr_meter : Subsystem
  sequences_data : Subsystem
  m : Outport
  wires:
  Bus Creator/1 -> m/1
  sequences_data/1(m_seq) -> Bus Creator/1  "sequences_data"
  pwr_meter/1(m_pwr_meter) -> Bus Creator/2  "pwr_meter"
  inner_current_tracking/1(m_inner_current_tracking) -> Bus Creator/3  "m_inner_current_tracking"
  [local_time] -> Bus Creator/5  "local_time"
  dq_pll/1(dqPLLs) -> Bus Creator/4  "dq_pll"

== system afe_inv_psm_param/afe_abc_inv_psm_mod1/AFE_control/afe_control/grid_current_sequences_and_reactive_pwr_ctrl ==
  ig_abc_pu : Inport
  current_sequence_avg : Subsystem
  grid_current_sampling_and_alpha_beta_transformation : Subsystem
  i_alphabeta2xieta : Subsystem
  sequences_current_control : Subsystem
  tag scope: i_grid_neg_eta_avg=scoped, i_grid_neg_xi_avg=scoped, i_grid_pos_eta_avg=scoped, i_grid_pos_xi_avg=scoped
  wires:
  i_alphabeta2xieta/1(xi) -> current_sequence_avg/1(i_grid_pos_xi)
  i_alphabeta2xieta/3(v_grid_neg_xi) -> current_sequence_avg/3(i_grid_neg_xi)
  i_alphabeta2xieta/4(e) -> current_sequence_avg/4(i_grid_neg_eta)
  current_sequence_avg/4(i_grid_neg_eta_avg) -> sequences_current_control/4(i_neg_eta), [i_grid_neg_eta_avg]
  ig_abc_pu/1 -> grid_current_sampling_and_alpha_beta_transformation/1(ig_abc)
  i_alphabeta2xieta/2(v_grid_pos_eta) -> current_sequence_avg/2(i_grid_pos_eta)
  current_sequence_avg/1(i_grid_pos_xi_avg) -> [i_grid_pos_xi_avg], sequences_current_control/1(i_pos_xi)
  current_sequence_avg/2(i_grid_pos_eta_avg) -> [i_grid_pos_eta_avg], sequences_current_control/2(i_pos_eta)
  [phase_grid_pll] -> i_alphabeta2xieta/3(gamma)
  grid_current_sampling_and_alpha_beta_transformation/2(i_grid_beta) -> i_alphabeta2xieta/2(beta)
  grid_current_sampling_and_alpha_beta_transformation/1(i_grid_alpha) -> i_alphabeta2xieta/1(alpha)
  current_sequence_avg/3(i_grid_neg_xi_avg) -> sequences_current_control/3(i_neg_xi), [i_grid_neg_xi_avg]

== system afe_inv_psm_param/afe_abc_inv_psm_mod1/AFE_control/afe_control/grid_phase_acquisition ==
  grid_phase : Inport
  Quantizer : Quantizer  QuantizationInterval=param.meas.adc_quantization
  Unit Delay : UnitDelay  SampleTime=-1
  Zero-Order Hold : ZeroOrderHold  SampleTime=-1
  grid_phased : Outport
  wires:
  Zero-Order Hold/1 -> Quantizer/1
  Unit Delay/1 -> grid_phased/1
  grid_phase/1 -> Zero-Order Hold/1
  Quantizer/1 -> Unit Delay/1

== system afe_inv_psm_param/afe_abc_inv_psm_mod1/AFE_control/afe_control/grid_voltage_phase_lock_loops ==
  ug_abc_pu : Inport
  Bus Creator : BusCreator  Inputs=5
  Bus Creator1 : BusCreator  Inputs=4
  Bus Creator2 : BusCreator  Inputs=2
  FHT-PLL : Subsystem
  FHT-PLL performance : Scope  NumInputPorts=2
      settings: ActiveDisplayYMinimum=-1.251220703125  ActiveDisplayYMaximum=1.251220703125  DataLoggingVariableName=ScopeData8
  FHT-PLL_simulink : Subsystem
  Variant Source1 : VariantSource  VariantControls={param.afe.pll.use_dq_pll_mode1 == 1, param.afe.pll.use_dq_pll_mode2 == 1, param.afe.pll.use_dq_pll_mode3 == 1, param.afe.pll.use_dq_pll_mode4 == 1}
  Variant Source2 : VariantSource  VariantControls={param.afe.pll.use_dq_pll_mode1 == 1, param.afe.pll.use_dq_pll_mode2 == 1, param.afe.pll.use_dq_pll_mode3 == 1, param.afe.pll.use_dq_pll_mode4 == 1}
  dq_pll : Subsystem
  dq_pll_ccaller : Subsystem
  dqpll_ccaler : Scope  NumInputPorts=3
      settings: ActiveDisplayYMinimum=-0.88802937790751446  ActiveDisplayYMaximum=4.5431143753230572  DataLoggingVariableName=ScopeData4
  pll_performances : Scope  NumInputPorts=2
      settings: ActiveDisplayYMinimum=-3.9264641704366507  ActiveDisplayYMaximum=3.9264746341683896  DataLoggingVariableName=ScopeData34
  tag scope: omega_grid_dqpll_ccaller=scoped, omega_grid_fht_simulink_pll=scoped, omega_grid_fhtsr_dqpll=scoped, omega_grid_pll_pu=scoped, omega_grid_pu_dqpll=scoped, phase_grid_dqpll=scoped, phase_grid_dqpll_ccaller=scoped, phase_grid_fht_simulink_pll=scoped, phase_grid_fhtsr_dqpll=scoped, phase_grid_pll=scoped
  wires:
  Variant Source1/1 -> [phase_grid_pll]
  FHT-PLL_simulink/1(gamma_grid_fht_pll) -> [phase_grid_fht_simulink_pll]
  FHT-PLL_simulink/2(omega_grid_fht_pll) -> [omega_grid_fht_simulink_pll]
  dq_pll/2(omega_grid_pu_dqpll) -> [omega_grid_pu_dqpll]
  dq_pll/1(phase_grid_dqpll) -> [phase_grid_dqpll]
  dq_pll_ccaller/1(gamma_hat) -> [phase_grid_dqpll_ccaller]
  dq_pll_ccaller/2(omega_pu_hat) -> [omega_grid_dqpll_ccaller]
  [phase_grid_dqpll] -> Variant Source1/1, Bus Creator/1  "phase_grid_dqpll"
  [phase_grid_dqpll_ccaller] -> Bus Creator/2, Variant Source1/2  "phase_grid_dqpll_ccaller"
  [phase_grid_fht_simulink_pll] -> Bus Creator/3, Variant Source1/3  "phase_grid_fht_simulink_pll"
  [omega_grid_pu_dqpll] -> Variant Source2/1, Bus Creator1/1  "omega_grid_pu_dqpll"
  [omega_grid_dqpll_ccaller] -> Variant Source2/2, Bus Creator1/2  "omega_grid_dqpll_ccaller"
  [omega_grid_fht_simulink_pll] -> Variant Source2/3, Bus Creator1/3  "omega_grid_fht_simulink_pll"
  Variant Source2/1 -> [omega_grid_pll_pu]
  dq_pll_ccaller/3(dqpll_uxi) -> dqpll_ccaler/1  "uxi_n"
  dq_pll_ccaller/4(dqpll_ueta) -> dqpll_ccaler/2  "ueta_n"
  dq_pll_ccaller/5(dqpll_state) -> dqpll_ccaler/3  "dqpll_state"
  ug_abc_pu/1 -> FHT-PLL performance/1, dq_pll/1(ug_abc_pu), FHT-PLL_simulink/1(ug_abc_pu), FHT-PLL/1(ug_abc_pu), dq_pll_ccaller/1(ug_abc_pu)
  Bus Creator/1 -> pll_performances/1
  Bus Creator1/1 -> pll_performances/2
  [grid_emulator_phase] -> Bus Creator/4  "grid_emulator_phase"
  FHT-PLL/2(omega_grid_fht_pll) -> [omega_grid_fhtsr_dqpll]
  FHT-PLL/1(gamma_grid_fht_pll) -> [phase_grid_fhtsr_dqpll]
  [phase_grid_fhtsr_dqpll] -> Bus Creator/5  "phase_grid_fht_pll"
  [omega_grid_fhtsr_dqpll] -> Bus Creator1/4  "omega_grid_fht_pll"
  [phase_grid_fhtsr_dqpll] -> Variant Source1/4  "phase_grid_fht_pll"
  [omega_grid_fhtsr_dqpll] -> Variant Source2/4  "omega_grid_fht_pll"
  Bus Creator2/1 -> FHT-PLL performance/2
  [omega_grid_fhtsr_dqpll] -> Bus Creator2/2  "omega_grid_fht_pll"
  [phase_grid_fhtsr_dqpll] -> Bus Creator2/1  "phase_grid_fht_pll"

== system afe_inv_psm_param/afe_abc_inv_psm_mod1/AFE_control/afe_control/grid_voltage_sequences ==
  grid_voltage_sampling_and_alpha_beta_transformation : Subsystem
  v_alphabeta2xieta : Subsystem
  voltage_sequence_avg : Subsystem
  tag scope: ug_alpha_pu=scoped, ug_beta_pu=scoped, v_grid_neg_eta_avg=scoped, v_grid_neg_xi_avg=scoped, v_grid_pos_eta_avg=scoped, v_grid_pos_xi_avg=scoped
  wires:
  v_alphabeta2xieta/4(v_grid_neg_eta) -> voltage_sequence_avg/4(v_grid_neg_eta)  "neg_eta"
  v_alphabeta2xieta/2(eta) -> voltage_sequence_avg/2(v_grid_pos_eta)  "pos_eta"
  [phase_grid_pll] -> v_alphabeta2xieta/3(gamma)
  v_alphabeta2xieta/3(v_grid_neg_xi) -> voltage_sequence_avg/3(v_grid_neg_xi)  "neg_xi"
  voltage_sequence_avg/3(v_grid_neg_xi_avg) -> [v_grid_neg_xi_avg]
  voltage_sequence_avg/2(v_grid_pos_eta_avg) -> [v_grid_pos_eta_avg]
  voltage_sequence_avg/4(v_grid_neg_eta_avg) -> [v_grid_neg_eta_avg]
  grid_voltage_sampling_and_alpha_beta_transformation/2(u_grid_beta) -> [ug_beta_pu], v_alphabeta2xieta/2(beta)
  voltage_sequence_avg/1(v_grid_pos_xi_avg) -> [v_grid_pos_xi_avg]
  v_alphabeta2xieta/1(xi) -> voltage_sequence_avg/1(v_grid_pos_xi)  "pos_xi"
  grid_voltage_sampling_and_alpha_beta_transformation/1(u_grid_alpha) -> [ug_alpha_pu], v_alphabeta2xieta/1(alpha)
  [ugd_abc_pu] -> grid_voltage_sampling_and_alpha_beta_transformation/1(v_abc)

== system afe_inv_psm_param/afe_abc_inv_psm_mod1/AFE_control/afe_control/i_xi_ref ==
  Constant1 : Constant  Value=param.afe.ref.ixi_ref_mod1
  Constant2 : Constant  Value=0
  Delay : Delay  DelayLength=floor(0.25/param.glb_time.ts_afe)
  Switch : Switch  Criteria=u2 > Threshold  SaturateOnIntegerOverflow=off  InputSameDT=off
  Switch1 : Switch  Criteria=u2 > Threshold  SaturateOnIntegerOverflow=off  InputSameDT=off
  Variant Source : VariantSource  VariantControls={false, true}
  discrete-time-low-pass-filter : discrete_time_low_pass_filter/discrete-time-low-pass-filter  tau=0.125  ts=param.glb_time.ts_afe
  i_xi_ref : Outport
  wires:
  Constant1/1 -> Switch/3  "i_xi_ref"
  Constant2/1 -> Switch/1
  [pwr_lim_enable] -> Switch/2
  [pwr_lim_enable] -> Delay/1
  Switch/1 -> discrete-time-low-pass-filter/1, Variant Source/2, Switch1/3
  Delay/1 -> Switch1/2
  discrete-time-low-pass-filter/1 -> Switch1/1
  Switch1/1 -> Variant Source/1
  Variant Source/1 -> i_xi_ref/1

== system afe_inv_psm_param/afe_abc_inv_psm_mod1/AFE_control/afe_control/ig afe quantizzation and one step delay ==
  ig_abc_pu : Inport
  Demux1 : Demux  Outputs=3
  Mux1 : Mux  Inputs=3
  ig afe quantizzation and one step delay : Subsystem
  igd_abc_pu : Outport
  wires:
  Demux1/1 -> ig afe quantizzation and one step delay/1(ig_u_pu)
  Demux1/2 -> ig afe quantizzation and one step delay/2(ig_v_pu)
  ig_abc_pu/1 -> Demux1/1
  Mux1/1 -> igd_abc_pu/1
  Demux1/3 -> ig afe quantizzation and one step delay/3(ig_w_pu)
  ig afe quantizzation and one step delay/2(igd_v_pu) -> Mux1/2
  ig afe quantizzation and one step delay/1(igd_u_pu) -> Mux1/1
  ig afe quantizzation and one step delay/3(igd_w_pu) -> Mux1/3

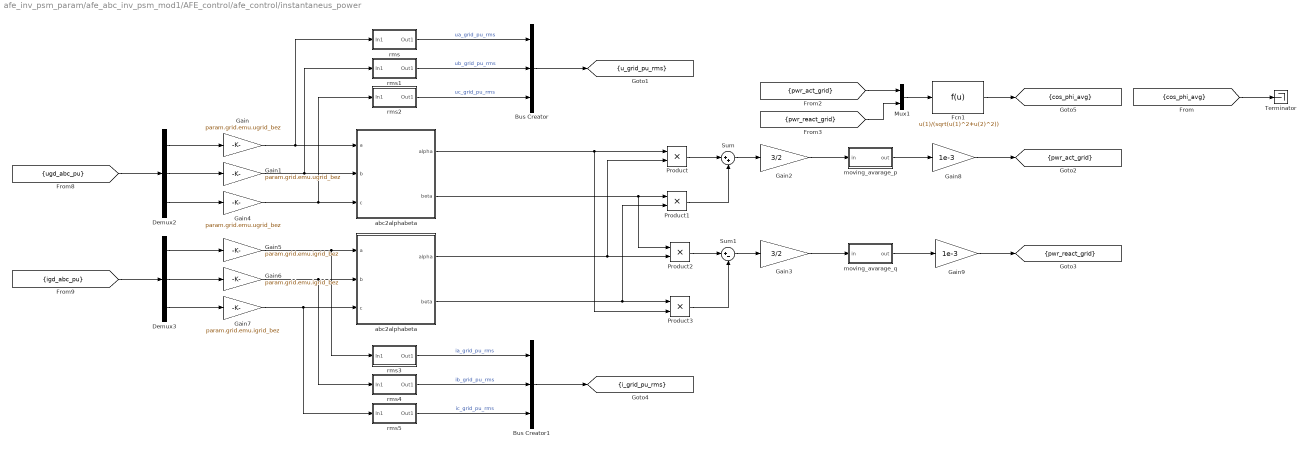
== system afe_inv_psm_param/afe_abc_inv_psm_mod1/AFE_control/afe_control/instantaneus_power ==
  Bus Creator : BusCreator  Inputs=3
  Bus Creator1 : BusCreator  Inputs=3
  Demux2 : Demux  Outputs=3
  Demux3 : Demux  Outputs=3
  Fcn1 : Fcn  Expr=u(1)/(sqrt(u(1)^2+u(2)^2))
  Gain : Gain  Gain=param.grid.emu.ugrid_bez
  Gain1 : Gain  Gain=param.grid.emu.ugrid_bez
  Gain2 : Gain  Gain=3/2
  Gain3 : Gain  Gain=3/2
  Gain4 : Gain  Gain=param.grid.emu.ugrid_bez
  Gain5 : Gain  Gain=param.grid.emu.igrid_bez
  Gain6 : Gain  Gain=param.grid.emu.igrid_bez
  Gain7 : Gain  Gain=param.grid.emu.igrid_bez
  Gain8 : Gain  Gain=1e-3
  Gain9 : Gain  Gain=1e-3
  Mux1 : Mux  Inputs=2
  Product{,1..3} (4 alike) : Product  RndMeth=Zero
  Sum : Sum  Inputs=|++
  Sum1 : Sum  Inputs=|+-
  Terminator : Terminator
  abc2alphabeta : Subsystem
  "abc2alphabeta " : Subsystem
  moving_avarage_p : Subsystem
  moving_avarage_q : Subsystem
  rms : Subsystem
  rms1 : Subsystem
  rms2 : Subsystem
  rms3 : Subsystem
  rms4 : Subsystem
  rms5 : Subsystem
  tag scope: cos_phi_avg=scoped, i_grid_pu_rms=scoped, pwr_act_grid=scoped, pwr_react_grid=scoped, u_grid_pu_rms=scoped
  wires:
  abc2alphabeta/2("beta ") -> Product1/1, Product2/1
  "abc2alphabeta "/2("beta ") -> Product1/2, Product3/1
  abc2alphabeta/1("alpha ") -> Product3/2, Product/1
  "abc2alphabeta "/1("alpha ") -> Product2/2, Product/2
  Product/1 -> Sum/1
  Product1/1 -> Sum/2
  Product2/1 -> Sum1/1
  Product3/1 -> Sum1/2
  Sum1/1 -> Gain3/1
  Sum/1 -> Gain2/1
  Gain2/1 -> moving_avarage_p/1(in)
  Gain3/1 -> moving_avarage_q/1(in)
  [pwr_react_grid] -> Mux1/2
  Mux1/1 -> Fcn1/1
  Fcn1/1 -> [cos_phi_avg]
  [pwr_act_grid] -> Mux1/1
  rms/1(Out1) -> Bus Creator/1  "ua_grid_pu_rms"
  rms2/1(Out1) -> Bus Creator/3  "uc_grid_pu_rms"
  rms1/1(Out1) -> Bus Creator/2  "ub_grid_pu_rms"
  moving_avarage_p/1(out) -> Gain8/1
  moving_avarage_q/1(out) -> Gain9/1
  Demux2/1 -> Gain/1
  Demux2/2 -> Gain1/1
  Demux2/3 -> Gain4/1
  Demux3/1 -> Gain5/1
  Demux3/2 -> Gain6/1
  Demux3/3 -> Gain7/1
  Gain/1 -> rms/1(In1), abc2alphabeta/1(a)
  Gain1/1 -> rms1/1(In1), abc2alphabeta/2(b)
  Gain4/1 -> rms2/1(In1), abc2alphabeta/3(c)
  Gain5/1 -> rms3/1(In1), "abc2alphabeta "/1(a)
  Gain6/1 -> rms4/1(In1), "abc2alphabeta "/2(b)
  Gain7/1 -> rms5/1(In1), "abc2alphabeta "/3(c)
  Gain8/1 -> [pwr_act_grid]
  Gain9/1 -> [pwr_react_grid]
  [ugd_abc_pu] -> Demux2/1
  [igd_abc_pu] -> Demux3/1
  Bus Creator/1 -> [u_grid_pu_rms]
  rms4/1(Out1) -> Bus Creator1/2  "ib_grid_pu_rms"
  rms3/1(Out1) -> Bus Creator1/1  "ia_grid_pu_rms"
  rms5/1(Out1) -> Bus Creator1/3  "ic_grid_pu_rms"
  Bus Creator1/1 -> [i_grid_pu_rms]
  [cos_phi_avg] -> Terminator/1

== system afe_inv_psm_param/afe_abc_inv_psm_mod1/AFE_control/afe_control/interesting scopes ==
  current_sequences_mod1 : Scope  NumInputPorts=4
      settings: ActiveDisplayYMinimum=-0.97178065031766891  ActiveDisplayYMaximum=1.9392475411295891  DataLoggingVariableName=ScopeData2
  i_grid_seq_ref : Scope
      settings: ActiveDisplayYMinimum=-1.1499999999999995  ActiveDisplayYMaximum=0.34999999999999981
  voltage_sequences_mod1 : Scope  NumInputPorts=4
      settings: ActiveDisplayYMinimum=-1.2405151816982258  ActiveDisplayYMaximum=1.2605257614333911
  wires:
  [v_grid_neg_eta_avg] -> voltage_sequences_mod1/4  "u_grid_neg_eta"
  [i_grid_neg_xi_avg] -> current_sequences_mod1/3  "i_grid_neg_xi"
  [v_grid_pos_eta_avg] -> voltage_sequences_mod1/2  "u_grid_pos_eta"
  [v_grid_neg_xi_avg] -> voltage_sequences_mod1/3  "u_grid_neg_xi"
  [i_grid_pos_xi_avg] -> current_sequences_mod1/1  "i_grid_pos_xi"
  [i_grid_neg_eta_avg] -> current_sequences_mod1/4  "i_grid_neg_eta"
  [v_grid_pos_xi_avg] -> voltage_sequences_mod1/1  "u_grid_pos_xi"
  [i_grid_pos_eta_avg] -> current_sequences_mod1/2  "i_grid_pos_eta"
  [i_grid_seq_ref] -> i_grid_seq_ref/1  "i_grid_seq_ref"

== system afe_inv_psm_param/afe_abc_inv_psm_mod1/AFE_control/afe_control/is afe quantizzation and one step delay ==
  is_abc_pu : Inport
  Demux : Demux  Outputs=3
  Mux : Mux  Inputs=3
  is afe quantizzation and one step delay : Subsystem
  isd_abc_pu : Outport
  wires:
  is afe quantizzation and one step delay/2(isd_v_pu) -> Mux/2
  is_abc_pu/1 -> Demux/1
  is afe quantizzation and one step delay/3(isd_w_pu) -> Mux/3
  is afe quantizzation and one step delay/1(isd_u_pu) -> Mux/1
  Demux/1 -> is afe quantizzation and one step delay/1(is_u_pu)
  Mux/1 -> isd_abc_pu/1
  Demux/3 -> is afe quantizzation and one step delay/3(is_w_pu)
  Demux/2 -> is afe quantizzation and one step delay/2(is_v_pu)

== system afe_inv_psm_param/afe_abc_inv_psm_mod1/AFE_control/afe_control/islanding_mode_detector ==
  gamma : Inport
  alpha : Inport  Port=2
  beta : Inport  Port=3
  Gain : Gain  Gain=7
  MATLAB Function : MATLAB Function  TreatAsAtomicUnit=on
  Terminator : Terminator
  Terminator1 : Terminator
  bounder : MATLAB Function  TreatAsAtomicUnit=on
  moving_avarage_1 : Subsystem
  moving_avarage_2 : Subsystem
  seventh_ugrid_component : Scope  NumInputPorts=2
      settings: ActiveDisplayYMinimum=-0.0034745064787606167  ActiveDisplayYMaximum=0.0074022094547510631  DataLoggingVariableName=ScopeData10
  tag scope: u_7th_eta_avg=scoped, u_7th_xi_avg=scoped
  wires:
  gamma/1 -> Gain/1  "gamma_grid"
  MATLAB Function/1(xi) -> moving_avarage_1/1(u)
  bounder/1(y) -> MATLAB Function/3(gamma)
  Gain/1 -> bounder/1(u)
  alpha/1 -> MATLAB Function/1(alpha)  "u_grid_alpha"
  beta/1 -> MATLAB Function/2(beta)  "u_grid_beta"
  MATLAB Function/2(eta) -> moving_avarage_2/1(u)
  moving_avarage_1/1(y) -> [u_7th_xi_avg], seventh_ugrid_component/1  "u_7th_xi"
  moving_avarage_2/1(y) -> [u_7th_eta_avg], seventh_ugrid_component/2  "u_7th_eta"
  [u_7th_xi_avg] -> Terminator/1
  [u_7th_eta_avg] -> Terminator1/1

== system afe_inv_psm_param/afe_abc_inv_psm_mod1/AFE_control/afe_control/phase_compensation_1 ==
  local_time : Inport
  master_time : Inport  Port=2
  Zero-Order Hold : ZeroOrderHold  SampleTime=-1
  Zero-Order Hold1 : ZeroOrderHold  SampleTime=-1
  alignment_eval_afe1 : Subsystem
  y : Outport
  wires:
  local_time/1 -> Zero-Order Hold/1
  master_time/1 -> Zero-Order Hold1/1
  alignment_eval_afe1/1(dp) -> y/1
  Zero-Order Hold/1 -> alignment_eval_afe1/1(local_time)
  Zero-Order Hold1/1 -> alignment_eval_afe1/2(master_time)

== system afe_inv_psm_param/afe_abc_inv_psm_mod1/AFE_control/afe_control/space_vector ==
  uab_out : Inport
  Bus Creator : BusCreator  Inputs=3
  Bus Selector : BusSelector  OutputSignals=da,db,dc
  Bus Selector1 : BusSelector  OutputSignals=ualpha_afe,ubeta_afe,ugamma_afe
  C Caller : CCaller  FunctionName=sv_pwm_cm_process_simulink  PortSpecificationStruct="%)30     .    B H   8    (     @         %    \"     8    !     0         %  0 \"0    $    _    07)G3F%M90  4&]R=$YA;64 4V-O<&4     26YD97@     5'EP90      4VEZ90      27-';&]B86P   X    P    !@    @    $          4    (     0    ,    !         !   P!O=70 #@   #     &    \"     0         !0    @    !     P    $         $  # &]U=  .    .     8    (    !          %    \"     $    &     0         0   ...(+3252 chars)"
  Constant : Constant  Value=param.glb_time.ts_afe
  Constant1 : Constant
  Data Type Conversion1 : DataTypeConversion  OutDataTypeStr=double  SaturateOnIntegerOverflow=off  RndMeth=Floor
  Data Type Conversion{4,15..16,18} (4 alike) : DataTypeConversion  OutDataTypeStr=single  SaturateOnIntegerOverflow=off  RndMeth=Floor
  Data Type Conversion17 : DataTypeConversion  OutDataTypeStr=uint32  SaturateOnIntegerOverflow=off  RndMeth=Floor
  Data Type Conversion2 : DataTypeConversion  OutDataTypeStr=double  SaturateOnIntegerOverflow=off  RndMeth=Floor
  Data Type Conversion3 : DataTypeConversion  OutDataTypeStr=double  SaturateOnIntegerOverflow=off  RndMeth=Floor
  Gain1 : Gain  Gain=sqrt(3)/2
  Gain2 : Gain  Gain=sqrt(3)/2
  Gain3 : Gain  Gain=param.afe.ref.u_cm_comp_mod1
  duvw : Outport
  wires:
  Data Type Conversion15/1 -> C Caller/2
  Bus Selector/2 -> Data Type Conversion2/1  "<db>"
  Data Type Conversion18/1 -> C Caller/1
  C Caller/1 -> Bus Selector/1
  Bus Creator/1 -> duvw/1
  Data Type Conversion1/1 -> Bus Creator/1  "du(k)"
  Bus Selector1/2 -> Gain2/1  "<ubeta_afe>"
  Bus Selector/3 -> Data Type Conversion3/1  "<dc>"
  Bus Selector1/1 -> Gain1/1  "<ualpha_afe>"
  Data Type Conversion2/1 -> Bus Creator/2  "dv(k)"
  Gain2/1 -> Data Type Conversion15/1
  Bus Selector/1 -> Data Type Conversion1/1  "<da>"
  Gain1/1 -> Data Type Conversion18/1
  Data Type Conversion3/1 -> Bus Creator/3  "dw(k)"
  Constant/1 -> Data Type Conversion16/1
  uab_out/1 -> Bus Selector1/1
  Constant1/1 -> Data Type Conversion17/1
  Data Type Conversion16/1 -> C Caller/4
  Data Type Conversion17/1 -> C Caller/5
  Bus Selector1/3 -> Gain3/1  "<ugamma_afe>"
  Gain3/1 -> Data Type Conversion4/1
  Data Type Conversion4/1 -> C Caller/3

== system afe_inv_psm_param/afe_abc_inv_psm_mod1/AFE_control/afe_control/udc_acquisition ==
  udc_pu : Inport
  Quantizer : Quantizer  QuantizationInterval=param.meas.adc_quantization
  Unit Delay : UnitDelay  SampleTime=-1
  Zero-Order Hold : ZeroOrderHold  SampleTime=-1
  udcd_pu : Outport
  wires:
  Quantizer/1 -> Unit Delay/1
  udc_pu/1 -> Zero-Order Hold/1
  Unit Delay/1 -> udcd_pu/1
  Zero-Order Hold/1 -> Quantizer/1
